simulink model "lab4"  (R2021b)
settings: Solver=VariableStepAuto  StartTime=0.0  StopTime=10.0  RelTol=1e-3
settings Model: Creator=13676840  LastModifiedBy=13676840

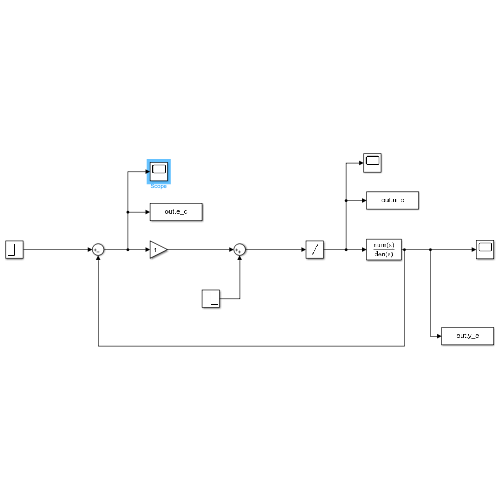
[thumbnail: Simulink's stored preview of the top-level diagram]
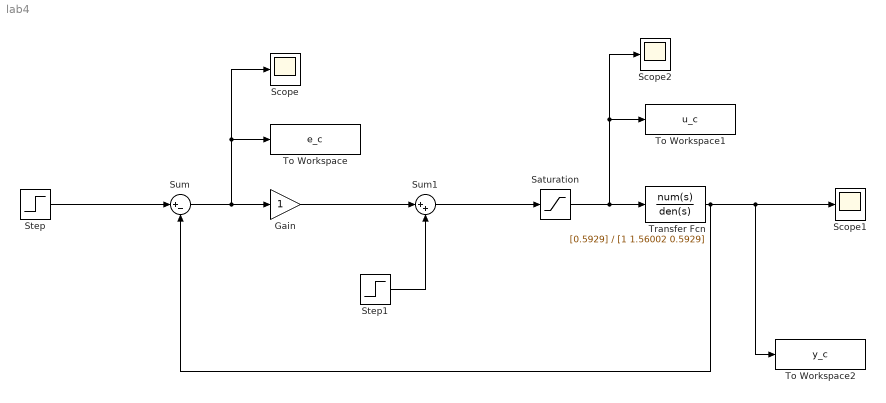
== system lab4 ==
  Gain : Gain
  Saturation : Saturate  UpperLimit=10  LowerLimit=-10
  Scope : Scope
  Scope1 : Scope
  Scope2 : Scope
  Step : Step  Time=0  After=1.17  SampleTime=0
  Step1 : Step  Time=12  After=-0.15  SampleTime=0
  Sum : Sum  Inputs=|+-
  Sum1 : Sum  Inputs=|++
  To Workspace : ToWorkspace  VariableName=e_c  SaveFormat=Timeseries  SampleTime=-1
  To Workspace1 : ToWorkspace  VariableName=u_c  SaveFormat=Timeseries  SampleTime=-1
  To Workspace2 : ToWorkspace  VariableName=y_c  SaveFormat=Timeseries  SampleTime=-1
  Transfer Fcn : TransferFcn  Numerator=[0.5929]  Denominator=[1 1.56002 0.5929]
  wires:
  Step/1 -> Sum/1
  Gain/1 -> Sum1/1
  Sum1/1 -> Saturation/1
  Saturation/1 -> To Workspace1/1, Scope2/1, Transfer Fcn/1
  Transfer Fcn/1 -> Sum/2, To Workspace2/1, Scope1/1
  Step1/1 -> Sum1/2
  Sum/1 -> To Workspace/1, Scope/1, Gain/1
